simulink model "AFC1_FFNN_trainrp_15_15_15_15_ep_1000_Nor_20250519"  (R2021a)
settings: Solver=ode15s  StartTime=0.0  StopTime=T  MaxStep=.01  RelTol=1e-3
undefined symbols (not defined in the file or in its folder): AF_sensor_tol, fault_time, fuel_inj_tol, kappa_tol, MAF_sensor_tol, pump_tol, tau_ww_tol, x_gain, x_offset, y_gain, y_offset
libraries: neural x66
(part 2 of 3)

== system AFC1_FFNN_trainrp_15_15_15_15_ep_1000_Nor_20250519/Air Fuel Control Model 1/Feed-Forward Neural Network/Layer 2/Delays 1 ==
  "p{2}" : Inport  PortDimensions=15
      mask Display: e = 0.06;c1 = [120 230 180]/255;c2 = ([120 230 180]+0)/(256+128);c3 = ([120 230 180]+128)/(256+128);patch([0 1 1 0],[0 0 1 1],c1);patch([0 1 1 1-e 1-e 0+e],[0 0 1 1-e 0+e 0+e],c2);patch([0 0 1 1-e 0+e 0+e],[0 1 1 1-e 1-e 0+e],c3);plot([0 1 1 0 0],[0 0 1 1 0]);
  mux : Mux  Inputs=1
      mask Display: e = 0.06;c1 = [120 150 230]/255;c2 = ([120 150 230]+0)/383;c3 = ([120 150 230]+128)/383;patch([0 1 1 0],[0 0 1 1],c1);patch([0 1 1 1-e 1-e 0+e],[0 0 1 1-e 0+e 0+e],c2);patch([0 0 1 1-e 0+e 0+e],[0 1 1 1-e 1-e 0+e],c3);plot([0 1 1 0 0],[0 0 1 1 0]);disp('Mux')
  "pd{2,1}" : Outport
      mask Display: e = 0.06;c1 = [120 230 180]/255;c2 = ([120 230 180]+0)/(256+128);c3 = ([120 230 180]+128)/(256+128);patch([0 1 1 0],[0 0 1 1],c1);patch([0 1 1 1-e 1-e 0+e],[0 0 1 1-e 0+e 0+e],c2);patch([0 0 1 1-e 0+e 0+e],[0 1 1 1-e 1-e 0+e],c3);plot([0 1 1 0 0],[0 0 1 1 0]);
  wires:
  mux/1 -> "pd{2,1}"/1
  "p{2}"/1 -> mux/1

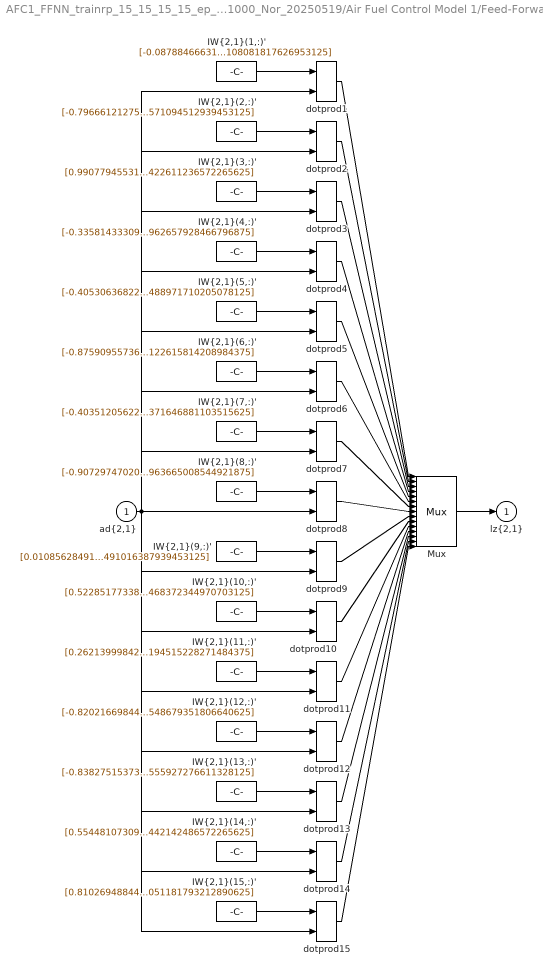
== system AFC1_FFNN_trainrp_15_15_15_15_ep_1000_Nor_20250519/Air Fuel Control Model 1/Feed-Forward Neural Network/Layer 2/LW{2,1} ==
  "ad{2,1}" : Inport  PortDimensions=15
      mask Display: e = 0.06;c1 = [120 230 180]/255;c2 = ([120 230 180]+0)/(256+128);c3 = ([120 230 180]+128)/(256+128);patch([0 1 1 0],[0 0 1 1],c1);patch([0 1 1 1-e 1-e 0+e],[0 0 1 1-e 0+e 0+e],c2);patch([0 0 1 1-e 0+e 0+e],[0 1 1 1-e 1-e 0+e],c3);plot([0 1 1 0 0],[0 0 1 1 0]);
  "IW{2,1}(1,:)'" : Constant  Value=[-0.0878846663125170124430951545946300029754638671875;0.252343903534000435495698866361635737121105194091796875;-0.1685271700099749969670170912650064565241336822509765625;-0.90573622777525797378217475852579809725284576416015625;0.4800646559755552544856982422061264514923095703125;-0.463888759594291821830580602181726135313510894775390625;-0.7754320756879466980393544872640632092952728271484375;0.2158502573908134269942138416809029877185821533203125;0.39940650684910306011943248449824750423431396484375;-0.29643323499838392098837402954814024269580841064453125;0.1823877518078674542234551836372702382504940032958984375;-0.1773465990403651770801474185645929537713527679443359375;-0.66625448256037433925058621753123588860034942626953125;-0.07347884281256167327001094236038625240325927734375;0.61840770258758670507859278586693108081817626953125]
      mask Display: e = 0.06;c1 = [120 150 230]/255;c2 = ([120 150 230]+0)/383;c3 = ([120 150 230]+128)/383;patch([0 1 1 0],[0 0 1 1],c1);patch([0 1 1 1-e 1-e 0+e],[0 0 1 1-e 0+e 0+e],c2);patch([0 0 1 1-e 0+e 0+e],[0 1 1 1-e 1-e 0+e],c3);plot([0 1 1 0 0],[0 0 1 1 0]);disp('weights');
  "IW{2,1}(10,:)'" : Constant  Value=[0.5228517733802267031251176376827061176300048828125;0.136935967661538982031999012178857810795307159423828125;-0.449953328272645391994188912576646544039249420166015625;-0.695014295696334105656433166586793959140777587890625;0.1958832707677782281052714097313582897186279296875;0.09859411313837000701010282455172273330390453338623046875;0.3109960796070747601760331235709600150585174560546875;-0.3914960581296071939760850000311620533466339111328125;-0.62009414863209888491013543898588977754116058349609375;1.0606054613447748469212683630757965147495269775390625;-1.5664825460309159677052548431674949824810028076171875;0.342344271691656210077070454644854180514812469482421875;0.5277958885729565619016057098633609712123870849609375;0.4054046139009506166672736071632243692874908447265625;-0.489226519023898465121646950137801468372344970703125]
      mask Display: e = 0.06;c1 = [120 150 230]/255;c2 = ([120 150 230]+0)/383;c3 = ([120 150 230]+128)/383;patch([0 1 1 0],[0 0 1 1],c1);patch([0 1 1 1-e 1-e 0+e],[0 0 1 1-e 0+e 0+e],c2);patch([0 0 1 1-e 0+e 0+e],[0 1 1 1-e 1-e 0+e],c3);plot([0 1 1 0 0],[0 0 1 1 0]);disp('weights');
  "IW{2,1}(11,:)'" : Constant  Value=[0.262139998427187048690711890230886638164520263671875;0.0522049315911223832387122456566430628299713134765625;0.0990802140303959077982653980143368244171142578125;0.2814358459318511140878626974881626665592193603515625;0.5787278872838108600973328066174872219562530517578125;-0.5952539605888416129886309136054478585720062255859375;-0.780489898553896832567033925442956387996673583984375;-0.438377123322267914229399821124388836324214935302734375;-0.8028118145780045455950357791152782738208770751953125;0.4134304353938611509278189259930513799190521240234375;-0.691260389041455258762880475842393934726715087890625;-0.350787364055528738671085875466815195977687835693359375;0.518654766262192534753694417304359376430511474609375;-0.692819246761199547535170495393685996532440185546875;-0.9589284506836308619170949896215461194515228271484375]
      mask Display: e = 0.06;c1 = [120 150 230]/255;c2 = ([120 150 230]+0)/383;c3 = ([120 150 230]+128)/383;patch([0 1 1 0],[0 0 1 1],c1);patch([0 1 1 1-e 1-e 0+e],[0 0 1 1-e 0+e 0+e],c2);patch([0 0 1 1-e 0+e 0+e],[0 1 1 1-e 1-e 0+e],c3);plot([0 1 1 0 0],[0 0 1 1 0]);disp('weights');
  "IW{2,1}(12,:)'" : Constant  Value=[-0.8202166984478165279170980284106917679309844970703125;0.274618896446455373894224294417654164135456085205078125;-0.09254118283008135048550713008808088488876819610595703125;-0.527171570486394625021375759388320147991180419921875;-0.26469416312424609571962719201110303401947021484375;-0.2440154859441432122491022482790867798030376434326171875;0.86751969677066487207639511325396597385406494140625;0.239684261725869429682234112988226115703582763671875;-1.021705503136143278197778272442519664764404296875;-0.1901820664902475754853838907365570776164531707763671875;-0.54306959111105612691972055472433567047119140625;-0.1891216002614057589692464489417034201323986053466796875;0.397296129957228461027085586465545929968357086181640625;0.90691413977249535349756115465424954891204833984375;0.8473512252408144096449404969462193548679351806640625]
      mask Display: e = 0.06;c1 = [120 150 230]/255;c2 = ([120 150 230]+0)/383;c3 = ([120 150 230]+128)/383;patch([0 1 1 0],[0 0 1 1],c1);patch([0 1 1 1-e 1-e 0+e],[0 0 1 1-e 0+e 0+e],c2);patch([0 0 1 1-e 0+e 0+e],[0 1 1 1-e 1-e 0+e],c3);plot([0 1 1 0 0],[0 0 1 1 0]);disp('weights');
  "IW{2,1}(13,:)'" : Constant  Value=[-0.8382751537393726692926065879873931407928466796875;0.414506970630843074587801311281509697437286376953125;0.73134430471062328305009714313200674951076507568359375;0.15362404519154726489915674392250366508960723876953125;-0.5879442809896107124956188272335566580295562744140625;-0.670655235646531622251131921075284481048583984375;-0.62507838715662700224129366688430309295654296875;0.89387205099974542665819399189786054193973541259765625;-125.13238631370819575749919749796390533447265625;-0.09474049935778734721214533465172280557453632354736328125;-1.2326114390598383874220189682091586291790008544921875;0.60217291030229247450478169412235729396343231201171875;0.4873766829746519757549094720161519944667816162109375;0.0817681624829529329900879019987769424915313720703125;0.3073997780165058646417719501187093555927276611328125]
      mask Display: e = 0.06;c1 = [120 150 230]/255;c2 = ([120 150 230]+0)/383;c3 = ([120 150 230]+128)/383;patch([0 1 1 0],[0 0 1 1],c1);patch([0 1 1 1-e 1-e 0+e],[0 0 1 1-e 0+e 0+e],c2);patch([0 0 1 1-e 0+e 0+e],[0 1 1 1-e 1-e 0+e],c3);plot([0 1 1 0 0],[0 0 1 1 0]);disp('weights');
  "IW{2,1}(14,:)'" : Constant  Value=[0.554481073097886412170964831602759659290313720703125;0.5627541035985543782516060673515312373638153076171875;0.5279205576257586240984664982534013688564300537109375;0.498262926207038159276407895958982408046722412109375;-0.8266669052089354874368609671364538371562957763671875;-0.259369160238817453301152227140846662223339080810546875;-0.4676423221847223476999033664469607174396514892578125;-0.7493356377816400293312426583725027740001678466796875;-0.6075021554860893235883168017608113586902618408203125;-0.737592874195698744443916439195163547992706298828125;0.516224862654837135522711832891218364238739013671875;-0.221330432748618688432173939872882328927516937255859375;-0.7881591665344693797834452198003418743610382080078125;0.3594677964209338494327994339982978999614715576171875;0.8652271440971281979415152818546630442142486572265625]
      mask Display: e = 0.06;c1 = [120 150 230]/255;c2 = ([120 150 230]+0)/383;c3 = ([120 150 230]+128)/383;patch([0 1 1 0],[0 0 1 1],c1);patch([0 1 1 1-e 1-e 0+e],[0 0 1 1-e 0+e 0+e],c2);patch([0 0 1 1-e 0+e 0+e],[0 1 1 1-e 1-e 0+e],c3);plot([0 1 1 0 0],[0 0 1 1 0]);disp('weights');
  "IW{2,1}(15,:)'" : Constant  Value=[0.810269488447141750242508351220749318599700927734375;-0.424046048771657524412148632109165191650390625;0.0119874076608134823296314408480611746199429035186767578125;0.1663714629097523545198100691777653992176055908203125;0.543867834198214605834209578461013734340667724609375;-0.66111839790786974813130427719443105161190032958984375;0.5956605204231941730341759466682560741901397705078125;-0.257123877719358129301241433495306409895420074462890625;-1326.833323485005166730843484401702880859375;0.2992922151314785228493065005750395357608795166015625;0.218990052974737670066218697684234939515590667724609375;-0.041318263947848064832069070462239324115216732025146484375;0.3631208609406313403411559193045832216739654541015625;-0.926873963903094288951933776843361556529998779296875;-0.6729752629449488043889004984521307051181793212890625]
      mask Display: e = 0.06;c1 = [120 150 230]/255;c2 = ([120 150 230]+0)/383;c3 = ([120 150 230]+128)/383;patch([0 1 1 0],[0 0 1 1],c1);patch([0 1 1 1-e 1-e 0+e],[0 0 1 1-e 0+e 0+e],c2);patch([0 0 1 1-e 0+e 0+e],[0 1 1 1-e 1-e 0+e],c3);plot([0 1 1 0 0],[0 0 1 1 0]);disp('weights');
  "IW{2,1}(2,:)'" : Constant  Value=[-0.7966612127504897333807321047061122953891754150390625;-0.59689157591508290590098795291851274669170379638671875;-0.11674709781591009749579512799755320884287357330322265625;-0.71982940180204779689887573113082908093929290771484375;-0.530346170504191416483763532596640288829803466796875;-0.132163879407860118675444027758203446865081787109375;0.5688557814878254514923128226655535399913787841796875;0.61984403455835879181989866992807947099208831787109375;-0.86428354009333252516711354473954997956752777099609375;-0.485260016390617276993424411557498387992382049560546875;-0.06465096978428530594129597375285811722278594970703125;0.45300372575796055141239548902376554906368255615234375;-0.86713196789925206520166511836578138172626495361328125;-0.5756735894901312544646998503594659268856048583984375;0.4972377435523942512674011595663614571094512939453125]
      mask Display: e = 0.06;c1 = [120 150 230]/255;c2 = ([120 150 230]+0)/383;c3 = ([120 150 230]+128)/383;patch([0 1 1 0],[0 0 1 1],c1);patch([0 1 1 1-e 1-e 0+e],[0 0 1 1-e 0+e 0+e],c2);patch([0 0 1 1-e 0+e 0+e],[0 1 1 1-e 1-e 0+e],c3);plot([0 1 1 0 0],[0 0 1 1 0]);disp('weights');
  "IW{2,1}(3,:)'" : Constant  Value=[0.9907794553101834100772293822956271469593048095703125;0.69361771571119656965009880877914838492870330810546875;-0.472958414836814944326448539868579246103763580322265625;-0.63814508065055919328045774818747304379940032958984375;0.4699150833921044156937796287820674479007720947265625;0.145553167558710672135902086665737442672252655029296875;-0.416859364186138225960576164652593433856964111328125;-1.108442454814500433002422141726128756999969482421875;0.80120742591300586621372303852695040404796600341796875;-0.363307602524073569583151765982620418071746826171875;-1.6971561491286279999002317708800546824932098388671875;-0.373394005260794636935628432183875702321529388427734375;-0.50362946973854560983596684309304691851139068603515625;-0.8029625246237832580931126358336769044399261474609375;-0.7596259640258387069167156369076110422611236572265625]
      mask Display: e = 0.06;c1 = [120 150 230]/255;c2 = ([120 150 230]+0)/383;c3 = ([120 150 230]+128)/383;patch([0 1 1 0],[0 0 1 1],c1);patch([0 1 1 1-e 1-e 0+e],[0 0 1 1-e 0+e 0+e],c2);patch([0 0 1 1-e 0+e 0+e],[0 1 1 1-e 1-e 0+e],c3);plot([0 1 1 0 0],[0 0 1 1 0]);disp('weights');
  "IW{2,1}(4,:)'" : Constant  Value=[-0.335814333095001860129968918045051395893096923828125;-0.3238045623956562479861531755886971950531005859375;-0.946818665892070754352971562184393405914306640625;0.5967017282279047929449689036118797957897186279296875;0.94119705017322896622999905957840383052825927734375;-0.612093495953800026398994305054657161235809326171875;0.207066877501773660696926526725292205810546875;-0.52412241175261886638736541499383747577667236328125;0.241146349875828669429012052205507643520832061767578125;0.7158448105719539267255413506063632667064666748046875;-0.276401362733712685493259186841896735131740570068359375;-0.008741392286228888419685745247988961637020111083984375;-0.3649588342015472886004090469214133918285369873046875;0.64714894785567711466001128428615629673004150390625;0.0500903295252175251306425707298330962657928466796875]
      mask Display: e = 0.06;c1 = [120 150 230]/255;c2 = ([120 150 230]+0)/383;c3 = ([120 150 230]+128)/383;patch([0 1 1 0],[0 0 1 1],c1);patch([0 1 1 1-e 1-e 0+e],[0 0 1 1-e 0+e 0+e],c2);patch([0 0 1 1-e 0+e 0+e],[0 1 1 1-e 1-e 0+e],c3);plot([0 1 1 0 0],[0 0 1 1 0]);disp('weights');
  "IW{2,1}(5,:)'" : Constant  Value=[-0.4053063682241566656472286922507919371128082275390625;-0.227253893947031937461389361487817950546741485595703125;0.472523309042105543742451345679000951349735260009765625;1.0204162791414053135241601921734400093555450439453125;0.7338605835038318758734021685086190700531005859375;0.392624606979962098574077344892430119216442108154296875;0.928845334431802616137474615243263542652130126953125;-0.81788247905176725272013982248608954250812530517578125;0.463839615645390057618868695499259047210216522216796875;0.511704719499542104443889911635778844356536865234375;-1.0401441393039692062671974781551398336887359619140625;0.7724822335363958902831882369355298578739166259765625;0.223380267932950238307654444724903441965579986572265625;-0.64998052523584082251772997551597654819488525390625;-0.3483327424735016553114519410883076488971710205078125]
      mask Display: e = 0.06;c1 = [120 150 230]/255;c2 = ([120 150 230]+0)/383;c3 = ([120 150 230]+128)/383;patch([0 1 1 0],[0 0 1 1],c1);patch([0 1 1 1-e 1-e 0+e],[0 0 1 1-e 0+e 0+e],c2);patch([0 0 1 1-e 0+e 0+e],[0 1 1 1-e 1-e 0+e],c3);plot([0 1 1 0 0],[0 0 1 1 0]);disp('weights');
  "IW{2,1}(6,:)'" : Constant  Value=[-0.8759095573607347251510191199486143887042999267578125;0.307826855407358712657384103295044042170047760009765625;-0.39001627189590981625855192760354839265346527099609375;0.06167114481671621961655915811206796206533908843994140625;-0.8275309402730073315979097969830036163330078125;-0.38639285520363919612663039515609852969646453857421875;-0.135030012059278003988538330304436385631561279296875;0.0940522282173063273180702026365906931459903717041015625;-0.231245412835122510220031699645915068686008453369140625;-0.1410617145612268197307770378756686113774776458740234375;0.45336813392401797973008115150150842964649200439453125;-0.160373216254841299832634149424848146736621856689453125;0.99787184814136808963525027138530276715755462646484375;-0.672860180430013610219930342282168567180633544921875;0.0928988798061369802638864712207578122615814208984375]
      mask Display: e = 0.06;c1 = [120 150 230]/255;c2 = ([120 150 230]+0)/383;c3 = ([120 150 230]+128)/383;patch([0 1 1 0],[0 0 1 1],c1);patch([0 1 1 1-e 1-e 0+e],[0 0 1 1-e 0+e 0+e],c2);patch([0 0 1 1-e 0+e 0+e],[0 1 1 1-e 1-e 0+e],c3);plot([0 1 1 0 0],[0 0 1 1 0]);disp('weights');
  "IW{2,1}(7,:)'" : Constant  Value=[-0.40351205622447228194005219847895205020904541015625;-0.979326763313207226957501916331239044666290283203125;0.215731814525891518741218533250503242015838623046875;-0.735834088572874467359952177503146231174468994140625;-0.2671267673616022353400012434576638042926788330078125;-0.6963089497674668226778749158256687223911285400390625;0.3895043892358802661846084447461180388927459716796875;-0.14087108149629390396739836432971060276031494140625;-0.782364123453909154903840317274443805217742919921875;-0.631132664484693517437108312151394784450531005859375;-0.19522333460767615775921512977220118045806884765625;-0.3293773385895077954188536750734783709049224853515625;0.8714617455697608594533676296123303472995758056640625;0.3319744328222211660062157534412108361721038818359375;-0.20223849523360204472055556834675371646881103515625]
      mask Display: e = 0.06;c1 = [120 150 230]/255;c2 = ([120 150 230]+0)/383;c3 = ([120 150 230]+128)/383;patch([0 1 1 0],[0 0 1 1],c1);patch([0 1 1 1-e 1-e 0+e],[0 0 1 1-e 0+e 0+e],c2);patch([0 0 1 1-e 0+e 0+e],[0 1 1 1-e 1-e 0+e],c3);plot([0 1 1 0 0],[0 0 1 1 0]);disp('weights');
  "IW{2,1}(8,:)'" : Constant  Value=[-0.90729747020363848974966458627022802829742431640625;-0.903105321493555823764154411037452518939971923828125;0.2073097679379041213820755729102529585361480712890625;0.5154490793135317883155721574439667165279388427734375;-0.2616023913399636580123797102714888751506805419921875;0.8353753633171170367432978309807367622852325439453125;0.5161985505789081773997395430342294275760650634765625;0.1632074331263788369295042457451927475631237030029296875;0.37370752723484113033691755845211446285247802734375;-0.314065206650639361374288682782207615673542022705078125;1.1214540191657054180041086510755121707916259765625;-0.133095776803223431183909042374580167233943939208984375;-0.084227332291266332475743183749727904796600341796875;0.7887787507084855764816211376455612480640411376953125;-0.16981322677390675579545131768099963665008544921875]
      mask Display: e = 0.06;c1 = [120 150 230]/255;c2 = ([120 150 230]+0)/383;c3 = ([120 150 230]+128)/383;patch([0 1 1 0],[0 0 1 1],c1);patch([0 1 1 1-e 1-e 0+e],[0 0 1 1-e 0+e 0+e],c2);patch([0 0 1 1-e 0+e 0+e],[0 1 1 1-e 1-e 0+e],c3);plot([0 1 1 0 0],[0 0 1 1 0]);disp('weights');
  "IW{2,1}(9,:)'" : Constant  Value=[0.010856284915405911561947505106218159198760986328125;0.151032243147247335901539599944953806698322296142578125;-0.8855070663425708143989822929142974317073822021484375;-0.7792930387153027549373973670299164950847625732421875;0.3700569453232185335167514494969509541988372802734375;-0.496699157187495632381768473351257853209972381591796875;-0.1347153477057989601206600127625279128551483154296875;0.52028451381425033783756362026906572282314300537109375;-0.9627013632476366655765787072596140205860137939453125;-0.60906020144285066830747155108838342130184173583984375;0.250323131030964873833255524004925973713397979736328125;0.206662192489482199331263245767331682145595550537109375;-0.60304320633583075039751975054969079792499542236328125;0.0331164167025408406885844669886864721775054931640625;-0.63852447949041124530822344240732491016387939453125]
      mask Display: e = 0.06;c1 = [120 150 230]/255;c2 = ([120 150 230]+0)/383;c3 = ([120 150 230]+128)/383;patch([0 1 1 0],[0 0 1 1],c1);patch([0 1 1 1-e 1-e 0+e],[0 0 1 1-e 0+e 0+e],c2);patch([0 0 1 1-e 0+e 0+e],[0 1 1 1-e 1-e 0+e],c3);plot([0 1 1 0 0],[0 0 1 1 0]);disp('weights');
  Mux : Mux  Inputs=15
      mask Display: e = 0.06;c1 = [120 150 230]/255;c2 = ([120 150 230]+0)/383;c3 = ([120 150 230]+128)/383;patch([0 1 1 0],[0 0 1 1],c1);patch([0 1 1 1-e 1-e 0+e],[0 0 1 1-e 0+e 0+e],c2);patch([0 0 1 1-e 0+e 0+e],[0 1 1 1-e 1-e 0+e],c3);plot([0 1 1 0 0],[0 0 1 1 0]);disp('Mux');
  dotprod{1..15} (15 alike) : neural/Weight Functions/dotprod
  "lz{2,1}" : Outport
      mask Display: e = 0.06;c1 = [120 230 180]/255;c2 = ([120 230 180]+0)/(256+128);c3 = ([120 230 180]+128)/(256+128);patch([0 1 1 0],[0 0 1 1],c1);patch([0 1 1 1-e 1-e 0+e],[0 0 1 1-e 0+e 0+e],c2);patch([0 0 1 1-e 0+e 0+e],[0 1 1 1-e 1-e 0+e],c3);plot([0 1 1 0 0],[0 0 1 1 0]);
  wires:
  Mux/1 -> "lz{2,1}"/1
  dotprod15/1 -> Mux/15
  "IW{2,1}(15,:)'"/1 -> dotprod15/1
  dotprod14/1 -> Mux/14
  "IW{2,1}(14,:)'"/1 -> dotprod14/1
  dotprod13/1 -> Mux/13
  "IW{2,1}(13,:)'"/1 -> dotprod13/1
  dotprod12/1 -> Mux/12
  "IW{2,1}(12,:)'"/1 -> dotprod12/1
  dotprod11/1 -> Mux/11
  "IW{2,1}(11,:)'"/1 -> dotprod11/1
  dotprod10/1 -> Mux/10
  "IW{2,1}(10,:)'"/1 -> dotprod10/1
  dotprod9/1 -> Mux/9
  "IW{2,1}(9,:)'"/1 -> dotprod9/1
  dotprod8/1 -> Mux/8
  "IW{2,1}(8,:)'"/1 -> dotprod8/1
  dotprod7/1 -> Mux/7
  "IW{2,1}(7,:)'"/1 -> dotprod7/1
  dotprod6/1 -> Mux/6
  "IW{2,1}(6,:)'"/1 -> dotprod6/1
  dotprod5/1 -> Mux/5
  "IW{2,1}(5,:)'"/1 -> dotprod5/1
  dotprod4/1 -> Mux/4
  "IW{2,1}(4,:)'"/1 -> dotprod4/1
  dotprod3/1 -> Mux/3
  "IW{2,1}(3,:)'"/1 -> dotprod3/1
  dotprod2/1 -> Mux/2
  "IW{2,1}(2,:)'"/1 -> dotprod2/1
  dotprod1/1 -> Mux/1
  "ad{2,1}"/1 -> dotprod15/2, dotprod14/2, dotprod13/2, dotprod12/2, dotprod11/2, dotprod10/2, dotprod9/2, dotprod8/2, dotprod7/2, dotprod6/2, dotprod5/2, dotprod4/2, dotprod3/2, dotprod2/2, dotprod1/2
  "IW{2,1}(1,:)'"/1 -> dotprod1/1

== system AFC1_FFNN_trainrp_15_15_15_15_ep_1000_Nor_20250519/Air Fuel Control Model 1/Feed-Forward Neural Network/Layer 3/Delays 1 ==
  "p{3}" : Inport  PortDimensions=15
      mask Display: e = 0.06;c1 = [120 230 180]/255;c2 = ([120 230 180]+0)/(256+128);c3 = ([120 230 180]+128)/(256+128);patch([0 1 1 0],[0 0 1 1],c1);patch([0 1 1 1-e 1-e 0+e],[0 0 1 1-e 0+e 0+e],c2);patch([0 0 1 1-e 0+e 0+e],[0 1 1 1-e 1-e 0+e],c3);plot([0 1 1 0 0],[0 0 1 1 0]);
  mux : Mux  Inputs=1
      mask Display: e = 0.06;c1 = [120 150 230]/255;c2 = ([120 150 230]+0)/383;c3 = ([120 150 230]+128)/383;patch([0 1 1 0],[0 0 1 1],c1);patch([0 1 1 1-e 1-e 0+e],[0 0 1 1-e 0+e 0+e],c2);patch([0 0 1 1-e 0+e 0+e],[0 1 1 1-e 1-e 0+e],c3);plot([0 1 1 0 0],[0 0 1 1 0]);disp('Mux')
  "pd{3,2}" : Outport
      mask Display: e = 0.06;c1 = [120 230 180]/255;c2 = ([120 230 180]+0)/(256+128);c3 = ([120 230 180]+128)/(256+128);patch([0 1 1 0],[0 0 1 1],c1);patch([0 1 1 1-e 1-e 0+e],[0 0 1 1-e 0+e 0+e],c2);patch([0 0 1 1-e 0+e 0+e],[0 1 1 1-e 1-e 0+e],c3);plot([0 1 1 0 0],[0 0 1 1 0]);
  wires:
  mux/1 -> "pd{3,2}"/1
  "p{3}"/1 -> mux/1

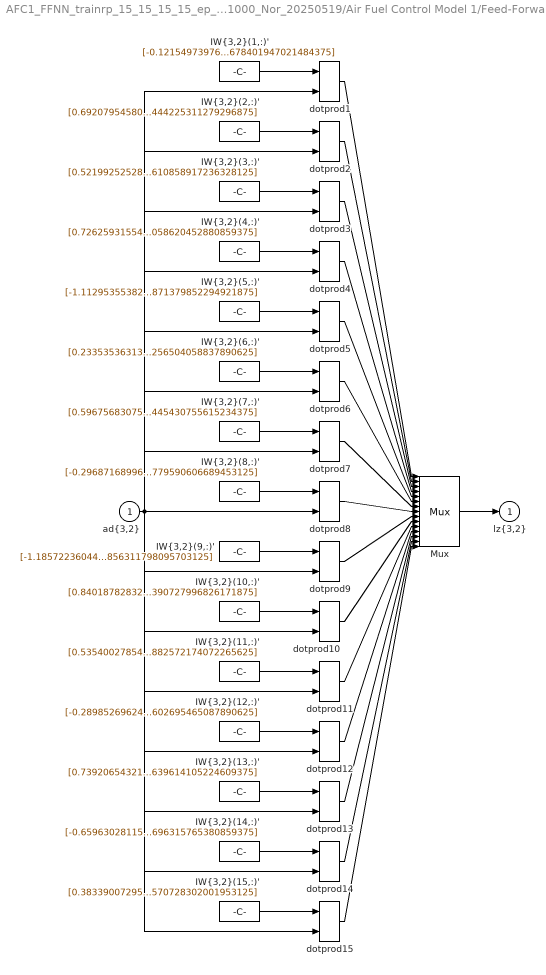
== system AFC1_FFNN_trainrp_15_15_15_15_ep_1000_Nor_20250519/Air Fuel Control Model 1/Feed-Forward Neural Network/Layer 3/LW{3,2} ==
  "ad{3,2}" : Inport  PortDimensions=15
      mask Display: e = 0.06;c1 = [120 230 180]/255;c2 = ([120 230 180]+0)/(256+128);c3 = ([120 230 180]+128)/(256+128);patch([0 1 1 0],[0 0 1 1],c1);patch([0 1 1 1-e 1-e 0+e],[0 0 1 1-e 0+e 0+e],c2);patch([0 0 1 1-e 0+e 0+e],[0 1 1 1-e 1-e 0+e],c3);plot([0 1 1 0 0],[0 0 1 1 0]);
  "IW{3,2}(1,:)'" : Constant  Value=[-0.12154973976904560883927075565225095488131046295166015625;0.2919742763312920263985006386064924299716949462890625;-2.0768198072644263874053649487905204296112060546875;0.55622562722152135705755426897667348384857177734375;1.0602287425168841483724690988310612738132476806640625;0.1906853701713702997633248514830484054982662200927734375;-0.17681297318493083281509825610555708408355712890625;0.66893230220344268577292723421123810112476348876953125;-0.7819647750905802663368149296729825437068939208984375;0.8737219689347257567391125121503137052059173583984375;0.002565826406430549155857079313136637210845947265625;0.59557072301141411596603347788914106786251068115234375;-0.1224255103849294645801393244255450554192066192626953125;0.390875932625203759140930515059153549373149871826171875;0.46442640116052602561325102215050719678401947021484375]
      mask Display: e = 0.06;c1 = [120 150 230]/255;c2 = ([120 150 230]+0)/383;c3 = ([120 150 230]+128)/383;patch([0 1 1 0],[0 0 1 1],c1);patch([0 1 1 1-e 1-e 0+e],[0 0 1 1-e 0+e 0+e],c2);patch([0 0 1 1-e 0+e 0+e],[0 1 1 1-e 1-e 0+e],c3);plot([0 1 1 0 0],[0 0 1 1 0]);disp('weights');
  "IW{3,2}(10,:)'" : Constant  Value=[0.84018782832057414822202190407551825046539306640625;0.55039916251996634510845751719898544251918792724609375;-76.0616960309171901144509320147335529327392578125;0.5388991672261400633914263380574993789196014404296875;0.333807564710129678342553916081669740378856658935546875;-0.1426078712170477380549726831304724328219890594482421875;0.9923122225937388574124042861512862145900726318359375;1.071368633560323413433934547356329858303070068359375;0.79479794213801080449144365047686733305454254150390625;0.0188693464052611704906414757942911819554865360260009765625;0.764987664832233793532623167266137897968292236328125;0.233017066036605491330391259907628409564495086669921875;0.2327832473727598772139657512525445781648159027099609375;-0.654474214960967248799761364352889358997344970703125;0.26373360138660373319652308055083267390727996826171875]
      mask Display: e = 0.06;c1 = [120 150 230]/255;c2 = ([120 150 230]+0)/383;c3 = ([120 150 230]+128)/383;patch([0 1 1 0],[0 0 1 1],c1);patch([0 1 1 1-e 1-e 0+e],[0 0 1 1-e 0+e 0+e],c2);patch([0 0 1 1-e 0+e 0+e],[0 1 1 1-e 1-e 0+e],c3);plot([0 1 1 0 0],[0 0 1 1 0]);disp('weights');
  "IW{3,2}(11,:)'" : Constant  Value=[0.53540027854651561778354107445920817553997039794921875;0.08451853867792070984510388598209829069674015045166015625;0.020898873773254035557389585164855816401541233062744140625;0.902208483791940185625435333349741995334625244140625;-0.3742391891738117148946685119881294667720794677734375;0.251263720798962364444406603070092387497425079345703125;-0.290931390086156316243659603060223162174224853515625;0.436257789100094661716155997055466286838054656982421875;-0.79964820614753173710909095461829565465450286865234375;0.755074763126760917231194980558939278125762939453125;0.4271480231886315426237388237495906651020050048828125;-0.3391527807867944499520262979785911738872528076171875;0.08802251178042695689551777604719973169267177581787109375;0.6734455634994349626509801964857615530490875244140625;-0.454203923295989631103708461523638106882572174072265625]
      mask Display: e = 0.06;c1 = [120 150 230]/255;c2 = ([120 150 230]+0)/383;c3 = ([120 150 230]+128)/383;patch([0 1 1 0],[0 0 1 1],c1);patch([0 1 1 1-e 1-e 0+e],[0 0 1 1-e 0+e 0+e],c2);patch([0 0 1 1-e 0+e 0+e],[0 1 1 1-e 1-e 0+e],c3);plot([0 1 1 0 0],[0 0 1 1 0]);disp('weights');
  "IW{3,2}(12,:)'" : Constant  Value=[-0.2898526962423020325587685874779708683490753173828125;-0.646289884749394527574395397095941007137298583984375;-0.9567003707393870737263341652578674256801605224609375;-0.940016099461220111521697617718018591403961181640625;-0.5643968125757508058626399360946379601955413818359375;-0.511669426419441464304327382706105709075927734375;0.9425176303668114652367648886865936219692230224609375;-0.9146802881299025411721004275023005902767181396484375;-0.6355449887978885659123307050322182476520538330078125;0.2578478773046357641618442357867024838924407958984375;0.2366747672438800353944543530815280973911285400390625;0.238943110355559706903250116738490760326385498046875;-0.5392338653650725621702122225542552769184112548828125;-0.7227965685152799579782367800362408161163330078125;0.3502248328102306462739079506718553602695465087890625]
      mask Display: e = 0.06;c1 = [120 150 230]/255;c2 = ([120 150 230]+0)/383;c3 = ([120 150 230]+128)/383;patch([0 1 1 0],[0 0 1 1],c1);patch([0 1 1 1-e 1-e 0+e],[0 0 1 1-e 0+e 0+e],c2);patch([0 0 1 1-e 0+e 0+e],[0 1 1 1-e 1-e 0+e],c3);plot([0 1 1 0 0],[0 0 1 1 0]);disp('weights');
  "IW{3,2}(13,:)'" : Constant  Value=[0.73920654321329537506102269617258571088314056396484375;0.65996804519144658396356817320338450372219085693359375;0.8911399770460570746166695244028232991695404052734375;0.07132838133447538808695753687061369419097900390625;-0.89051784821913260170589410336106084287166595458984375;-0.66378549833680644542965865184669382870197296142578125;-0.3071024773992807599398702222970314323902130126953125;-0.173627725899562268541131970778224058449268341064453125;-0.80880943515508307850581104503362439572811126708984375;-0.80393222237537564911491472230409272015094757080078125;-0.383424219517309150528916461553308181464672088623046875;-0.43272685799559462704877432770445011556148529052734375;0.16745710236065025622309576647239737212657928466796875;0.17641877077898726611238089390099048614501953125;-0.43195590161067831669328143107122741639614105224609375]
      mask Display: e = 0.06;c1 = [120 150 230]/255;c2 = ([120 150 230]+0)/383;c3 = ([120 150 230]+128)/383;patch([0 1 1 0],[0 0 1 1],c1);patch([0 1 1 1-e 1-e 0+e],[0 0 1 1-e 0+e 0+e],c2);patch([0 0 1 1-e 0+e 0+e],[0 1 1 1-e 1-e 0+e],c3);plot([0 1 1 0 0],[0 0 1 1 0]);disp('weights');
  "IW{3,2}(14,:)'" : Constant  Value=[-0.659630281150788366772985682473517954349517822265625;-0.045540028374880574257854704001147183589637279510498046875;2.47619536874311574337070851470343768596649169921875;-0.8258455601982153115869778048363514244556427001953125;-0.71804125368126248130096200839034281671047210693359375;0.251156742461004112154654421829036436975002288818359375;0.7730877235206126130151460529305040836334228515625;0.464651639945274030907285123248584568500518798828125;0.055309231616775568485255831774338730610907077789306640625;-0.132799948014607982482715442529297433793544769287109375;0.8720546533795394683608037666999734938144683837890625;0.47101908700388861461760825477540493011474609375;-0.87842003897898057740434296647435985505580902099609375;-0.267686399090124371724641605396755039691925048828125;2.63456914634946937070480998954735696315765380859375]
      mask Display: e = 0.06;c1 = [120 150 230]/255;c2 = ([120 150 230]+0)/383;c3 = ([120 150 230]+128)/383;patch([0 1 1 0],[0 0 1 1],c1);patch([0 1 1 1-e 1-e 0+e],[0 0 1 1-e 0+e 0+e],c2);patch([0 0 1 1-e 0+e 0+e],[0 1 1 1-e 1-e 0+e],c3);plot([0 1 1 0 0],[0 0 1 1 0]);disp('weights');
  "IW{3,2}(15,:)'" : Constant  Value=[0.383390072952821514551402515280642546713352203369140625;1.287347083378775014494976858259178698062896728515625;2.6939821150113925085634036804549396038055419921875;0.604182881111607894553117148461751639842987060546875;-0.4081722008125325817928796823252923786640167236328125;0.0206936608375957453720417333897785283625125885009765625;-0.09061027001618437992647159262560307979583740234375;0.6791267141624686143330791310290805995464324951171875;-0.2008731757276325524674831513038952834904193878173828125;-0.6429791531527022652170444416697137057781219482421875;-0.7504519186790148399524014166672714054584503173828125;-0.2071985026196206669535371247548027895390987396240234375;-1.9821421824674534395427372146514244377613067626953125;0.6135190893222113306393339371425099670886993408203125;3.940603862118198907893429350224323570728302001953125]
      mask Display: e = 0.06;c1 = [120 150 230]/255;c2 = ([120 150 230]+0)/383;c3 = ([120 150 230]+128)/383;patch([0 1 1 0],[0 0 1 1],c1);patch([0 1 1 1-e 1-e 0+e],[0 0 1 1-e 0+e 0+e],c2);patch([0 0 1 1-e 0+e 0+e],[0 1 1 1-e 1-e 0+e],c3);plot([0 1 1 0 0],[0 0 1 1 0]);disp('weights');
  "IW{3,2}(2,:)'" : Constant  Value=[0.692079545801302487006978481076657772064208984375;-0.162509137033730099997086426810710690915584564208984375;-0.2108723847147100649568329799876664765179157257080078125;-0.23338736274894156252912580384872853755950927734375;-0.803107483204499761342276542563922703266143798828125;0.9423220203221334134724429532070644199848175048828125;0.20527643607279433268786306143738329410552978515625;-0.63453586328539923755442941910587251186370849609375;-0.39889053645326988384312016933108679950237274169921875;-0.83682070063637092882657952941372059285640716552734375;-0.1365576562315056197149942818214185535907745361328125;0.35595486485162763923284501288435421884059906005859375;0.45248646626522026625849548508995212614536285400390625;-0.904890653772267850030175395659171044826507568359375;-0.0208113225532915446791548674809746444225311279296875]
      mask Display: e = 0.06;c1 = [120 150 230]/255;c2 = ([120 150 230]+0)/383;c3 = ([120 150 230]+128)/383;patch([0 1 1 0],[0 0 1 1],c1);patch([0 1 1 1-e 1-e 0+e],[0 0 1 1-e 0+e 0+e],c2);patch([0 0 1 1-e 0+e 0+e],[0 1 1 1-e 1-e 0+e],c3);plot([0 1 1 0 0],[0 0 1 1 0]);disp('weights');
  "IW{3,2}(3,:)'" : Constant  Value=[0.52199252528272699347411389680928550660610198974609375;-0.93454712348981783254231459068250842392444610595703125;-0.68778488127538828234008860817993991076946258544921875;0.164558464632898415747064291281276382505893707275390625;0.6837714583973169002462100252159871160984039306640625;-0.220192538065342280351188719578203745186328887939453125;0.5010401118474712145456351208849810063838958740234375;-0.6960522004228142378678967361338436603546142578125;1.28103643582833814917876225081272423267364501953125;-1.09097737267470318300865983474068343639373779296875;0.925120699024378101427146248170174658298492431640625;0.80070397133859005922573714997270144522190093994140625;0.56166644570993096152733414783142507076263427734375;-0.372430382979882235172652826804551295936107635498046875;-0.132088353331665075973688772137393243610858917236328125]
      mask Display: e = 0.06;c1 = [120 150 230]/255;c2 = ([120 150 230]+0)/383;c3 = ([120 150 230]+128)/383;patch([0 1 1 0],[0 0 1 1],c1);patch([0 1 1 1-e 1-e 0+e],[0 0 1 1-e 0+e 0+e],c2);patch([0 0 1 1-e 0+e 0+e],[0 1 1 1-e 1-e 0+e],c3);plot([0 1 1 0 0],[0 0 1 1 0]);disp('weights');
  "IW{3,2}(4,:)'" : Constant  Value=[0.7262593155473704431557280258857645094394683837890625;-0.80627796905046522635274186541209928691387176513671875;-327.03923681191503192167147062718868255615234375;0.1509897194056277758278383771539665758609771728515625;-0.84162783833373489006390855138306505978107452392578125;-0.34674181988097207973709146244800649583339691162109375;0.1670663485239172185714551233104430139064788818359375;1.6580351134444466509876292548142373561859130859375;-0.042442468164096198990353769886496593244373798370361328125;0.2127481472470130474672345144426799379289150238037109375;0.623205161990645795100363102392293512821197509765625;-0.133435543562449077104048456021700985729694366455078125;2.623567994574135919805257799453102052211761474609375;-0.167318839288513598884122757226577959954738616943359375;-1.304720301003170046527657177648507058620452880859375]
      mask Display: e = 0.06;c1 = [120 150 230]/255;c2 = ([120 150 230]+0)/383;c3 = ([120 150 230]+128)/383;patch([0 1 1 0],[0 0 1 1],c1);patch([0 1 1 1-e 1-e 0+e],[0 0 1 1-e 0+e 0+e],c2);patch([0 0 1 1-e 0+e 0+e],[0 1 1 1-e 1-e 0+e],c3);plot([0 1 1 0 0],[0 0 1 1 0]);disp('weights');
  "IW{3,2}(5,:)'" : Constant  Value=[-1.112953553822887631241655981284566223621368408203125;-0.386458830852877355255259317345917224884033203125;-0.92436622449378325061530858874903060495853424072265625;-0.009896590469968769010478126801899634301662445068359375;0.138993889109350676758225517914979718625545501708984375;0.6226188339689031625567849914659745991230010986328125;0.1035850298719349638076892006210982799530029296875;0.277089471329663605825288641426595859229564666748046875;-1.2307929217319948378417393541894853115081787109375;0.3163067959918881566494519574916921555995941162109375;-0.0286966602039646634381142575875855982303619384765625;0.314844418721271834815667034490616060793399810791015625;0.261500203981151313481490205958834849298000335693359375;-0.518190005759778582472563357441686093807220458984375;-1.025066760776503382857072210754267871379852294921875]
      mask Display: e = 0.06;c1 = [120 150 230]/255;c2 = ([120 150 230]+0)/383;c3 = ([120 150 230]+128)/383;patch([0 1 1 0],[0 0 1 1],c1);patch([0 1 1 1-e 1-e 0+e],[0 0 1 1-e 0+e 0+e],c2);patch([0 0 1 1-e 0+e 0+e],[0 1 1 1-e 1-e 0+e],c3);plot([0 1 1 0 0],[0 0 1 1 0]);disp('weights');
  "IW{3,2}(6,:)'" : Constant  Value=[0.233535363139929008635675700134015642106533050537109375;-0.52347538735295151557380677331821061670780181884765625;-0.0707948054941314186550016529508866369724273681640625;-0.44986048835612990615118178538978099822998046875;0.49018244712652592198764978093095123767852783203125;0.70635837807052526127193914362578652799129486083984375;0.1671412375154288643130939817638136446475982666015625;0.345075847094594490016561394440941512584686279296875;1.461986965021789597329870957764796912670135498046875;-0.41608281107720890279466630090610124170780181884765625;0.7888955111347863979887051755213178694248199462890625;0.48564102095626104915737641931627877056598663330078125;0.112076750107975520176495365376467816531658172607421875;0.360090026592353062984130929180537350475788116455078125;1.0266498004751980488435947336256504058837890625]
      mask Display: e = 0.06;c1 = [120 150 230]/255;c2 = ([120 150 230]+0)/383;c3 = ([120 150 230]+128)/383;patch([0 1 1 0],[0 0 1 1],c1);patch([0 1 1 1-e 1-e 0+e],[0 0 1 1-e 0+e 0+e],c2);patch([0 0 1 1-e 0+e 0+e],[0 1 1 1-e 1-e 0+e],c3);plot([0 1 1 0 0],[0 0 1 1 0]);disp('weights');
  "IW{3,2}(7,:)'" : Constant  Value=[0.596756830756270506554983512614853680133819580078125;0.2311905349389062613862932948904926888644695281982421875;0.5163469583661906003868580228299833834171295166015625;-0.5027420806760591887041300651617348194122314453125;-0.0916048642345434760425604281408595852553844451904296875;0.346289356867078346180477410598541609942913055419921875;0.02363983991695040032254837569780647754669189453125;-0.0391447700262055608977362908262875862419605255126953125;-0.950784491003366927230899818823672831058502197265625;-0.9470670413713297985935923861688934266567230224609375;-0.79490681046587052804852646659128367900848388671875;-0.32007920527548117117788706309511326253414154052734375;0.90134891275908624042045858004712499678134918212890625;0.7123645840125758521566012859693728387355804443359375;-1.254204404170914610716636161669157445430755615234375]
      mask Display: e = 0.06;c1 = [120 150 230]/255;c2 = ([120 150 230]+0)/383;c3 = ([120 150 230]+128)/383;patch([0 1 1 0],[0 0 1 1],c1);patch([0 1 1 1-e 1-e 0+e],[0 0 1 1-e 0+e 0+e],c2);patch([0 0 1 1-e 0+e 0+e],[0 1 1 1-e 1-e 0+e],c3);plot([0 1 1 0 0],[0 0 1 1 0]);disp('weights');
  "IW{3,2}(8,:)'" : Constant  Value=[-0.296871689962379281535476138742524199187755584716796875;-0.444074626969603813986253726397990249097347259521484375;-0.489924708836419753321678172142128460109233856201171875;-0.0967224590960544805540166635182686150074005126953125;0.58591890186228356984798892881372012197971343994140625;0.79180452462657247014732320167240686714649200439453125;-0.8348145460026012987242438612156547605991363525390625;-1.0503954954738758953425303843687288463115692138671875;0.57528677139516914973427219592849723994731903076171875;-0.5068886435045636407181746108108200132846832275390625;-0.2199901711094292000581162938033230602741241455078125;-0.08027676628329009911322344805739703588187694549560546875;-1.1209547409920432858854155711014755070209503173828125;-0.4369846097628933279111151932738721370697021484375;0.86191666828126944910337670080480165779590606689453125]
      mask Display: e = 0.06;c1 = [120 150 230]/255;c2 = ([120 150 230]+0)/383;c3 = ([120 150 230]+128)/383;patch([0 1 1 0],[0 0 1 1],c1);patch([0 1 1 1-e 1-e 0+e],[0 0 1 1-e 0+e 0+e],c2);patch([0 0 1 1-e 0+e 0+e],[0 1 1 1-e 1-e 0+e],c3);plot([0 1 1 0 0],[0 0 1 1 0]);disp('weights');
  "IW{3,2}(9,:)'" : Constant  Value=[-1.1857223604410480621851320393034256994724273681640625;0.2322081749364122149614786394522525370121002197265625;0.136433649005807622334174311617971397936344146728515625;-0.5445743479469047354513122627395205199718475341796875;0.3470977978122802287685999544919468462467193603515625;0.227902774433188515246229144395329058170318603515625;0.4391402697189794590570954824215732514858245849609375;0.686426676021019144258161759353242814540863037109375;0.2280833358705296465274159345426596701145172119140625;-1.03062072591289588530116816400550305843353271484375;0.854712449996249734596176494960673153400421142578125;0.65249826486778428336066326664877124130725860595703125;-0.7371740276349159071145322741358540952205657958984375;0.46210165944748293753718826337717473506927490234375;-0.789586313755247903856115954113192856311798095703125]
      mask Display: e = 0.06;c1 = [120 150 230]/255;c2 = ([120 150 230]+0)/383;c3 = ([120 150 230]+128)/383;patch([0 1 1 0],[0 0 1 1],c1);patch([0 1 1 1-e 1-e 0+e],[0 0 1 1-e 0+e 0+e],c2);patch([0 0 1 1-e 0+e 0+e],[0 1 1 1-e 1-e 0+e],c3);plot([0 1 1 0 0],[0 0 1 1 0]);disp('weights');
  Mux : Mux  Inputs=15
      mask Display: e = 0.06;c1 = [120 150 230]/255;c2 = ([120 150 230]+0)/383;c3 = ([120 150 230]+128)/383;patch([0 1 1 0],[0 0 1 1],c1);patch([0 1 1 1-e 1-e 0+e],[0 0 1 1-e 0+e 0+e],c2);patch([0 0 1 1-e 0+e 0+e],[0 1 1 1-e 1-e 0+e],c3);plot([0 1 1 0 0],[0 0 1 1 0]);disp('Mux');
  dotprod{1..15} (15 alike) : neural/Weight Functions/dotprod
  "lz{3,2}" : Outport
      mask Display: e = 0.06;c1 = [120 230 180]/255;c2 = ([120 230 180]+0)/(256+128);c3 = ([120 230 180]+128)/(256+128);patch([0 1 1 0],[0 0 1 1],c1);patch([0 1 1 1-e 1-e 0+e],[0 0 1 1-e 0+e 0+e],c2);patch([0 0 1 1-e 0+e 0+e],[0 1 1 1-e 1-e 0+e],c3);plot([0 1 1 0 0],[0 0 1 1 0]);
  wires:
  Mux/1 -> "lz{3,2}"/1
  dotprod15/1 -> Mux/15
  "IW{3,2}(15,:)'"/1 -> dotprod15/1
  dotprod14/1 -> Mux/14
  "IW{3,2}(14,:)'"/1 -> dotprod14/1
  dotprod13/1 -> Mux/13
  "IW{3,2}(13,:)'"/1 -> dotprod13/1
  dotprod12/1 -> Mux/12
  "IW{3,2}(12,:)'"/1 -> dotprod12/1
  dotprod11/1 -> Mux/11
  "IW{3,2}(11,:)'"/1 -> dotprod11/1
  dotprod10/1 -> Mux/10
  "IW{3,2}(10,:)'"/1 -> dotprod10/1
  dotprod9/1 -> Mux/9
  "IW{3,2}(9,:)'"/1 -> dotprod9/1
  dotprod8/1 -> Mux/8
  "IW{3,2}(8,:)'"/1 -> dotprod8/1
  dotprod7/1 -> Mux/7
  "IW{3,2}(7,:)'"/1 -> dotprod7/1
  dotprod6/1 -> Mux/6
  "IW{3,2}(6,:)'"/1 -> dotprod6/1
  dotprod5/1 -> Mux/5
  "IW{3,2}(5,:)'"/1 -> dotprod5/1
  dotprod4/1 -> Mux/4
  "IW{3,2}(4,:)'"/1 -> dotprod4/1
  dotprod3/1 -> Mux/3
  "IW{3,2}(3,:)'"/1 -> dotprod3/1
  dotprod2/1 -> Mux/2
  "IW{3,2}(2,:)'"/1 -> dotprod2/1
  dotprod1/1 -> Mux/1
  "ad{3,2}"/1 -> dotprod15/2, dotprod14/2, dotprod13/2, dotprod12/2, dotprod11/2, dotprod10/2, dotprod9/2, dotprod8/2, dotprod7/2, dotprod6/2, dotprod5/2, dotprod4/2, dotprod3/2, dotprod2/2, dotprod1/2
  "IW{3,2}(1,:)'"/1 -> dotprod1/1

== system AFC1_FFNN_trainrp_15_15_15_15_ep_1000_Nor_20250519/Air Fuel Control Model 1/Feed-Forward Neural Network/Layer 4/Delays 1 ==
  "p{4}" : Inport  PortDimensions=15
      mask Display: e = 0.06;c1 = [120 230 180]/255;c2 = ([120 230 180]+0)/(256+128);c3 = ([120 230 180]+128)/(256+128);patch([0 1 1 0],[0 0 1 1],c1);patch([0 1 1 1-e 1-e 0+e],[0 0 1 1-e 0+e 0+e],c2);patch([0 0 1 1-e 0+e 0+e],[0 1 1 1-e 1-e 0+e],c3);plot([0 1 1 0 0],[0 0 1 1 0]);
  mux : Mux  Inputs=1
      mask Display: e = 0.06;c1 = [120 150 230]/255;c2 = ([120 150 230]+0)/383;c3 = ([120 150 230]+128)/383;patch([0 1 1 0],[0 0 1 1],c1);patch([0 1 1 1-e 1-e 0+e],[0 0 1 1-e 0+e 0+e],c2);patch([0 0 1 1-e 0+e 0+e],[0 1 1 1-e 1-e 0+e],c3);plot([0 1 1 0 0],[0 0 1 1 0]);disp('Mux')
  "pd{4,3}" : Outport
      mask Display: e = 0.06;c1 = [120 230 180]/255;c2 = ([120 230 180]+0)/(256+128);c3 = ([120 230 180]+128)/(256+128);patch([0 1 1 0],[0 0 1 1],c1);patch([0 1 1 1-e 1-e 0+e],[0 0 1 1-e 0+e 0+e],c2);patch([0 0 1 1-e 0+e 0+e],[0 1 1 1-e 1-e 0+e],c3);plot([0 1 1 0 0],[0 0 1 1 0]);
  wires:
  mux/1 -> "pd{4,3}"/1
  "p{4}"/1 -> mux/1
